simulink model "heater"  (R2024a)
settings: Solver=VariableStepAuto  StartTime=0.0  StopTime=10.0  RelTol=1e-3
settings Model: Creator=raphg  LastModifiedBy=raphg

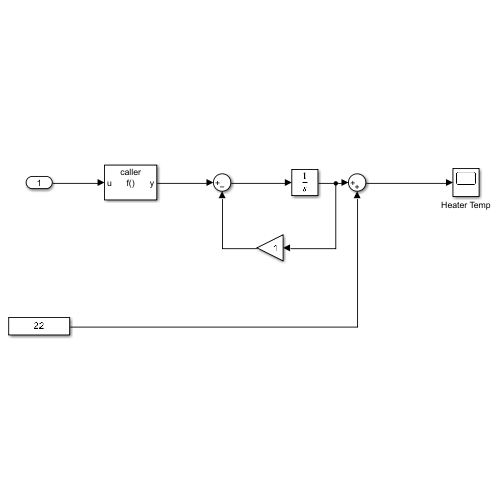
[thumbnail: Simulink's stored preview of the top-level diagram]
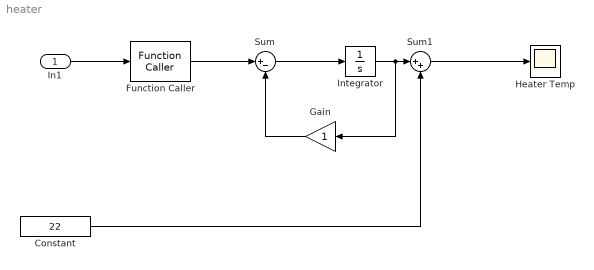
== system heater ==
  In1 : Inport
  Constant : Constant  Value=22
  Function Caller : FunctionCaller  FunctionPrototype=y = f(u)  InputArgumentSpecifications=<Enter example>  OutputArgumentSpecifications=<Enter example>
  Gain : Gain
  Heater Temp : Scope
  Integrator : Integrator
  Sum : Sum  Inputs=|+-
  Sum1 : Sum  Inputs=|++
  wires:
  Sum/1 -> Integrator/1
  In1/1 -> Function Caller/1
  Function Caller/1 -> Sum/1
  Integrator/1 -> Gain/1, Sum1/1
  Constant/1 -> Sum1/2
  Sum1/1 -> Heater Temp/1
  Gain/1 -> Sum/2
